simulink model "mavsim"  (R2025b)
settings: Solver=ode45  StartTime=0.0  StopTime=80  RelTol=1e-3
undefined symbols (not defined in the file): animation_block, autopilot_block, forces_block, P, wind_block
settings Model: Creator=parakh  LastModifiedBy=parakh

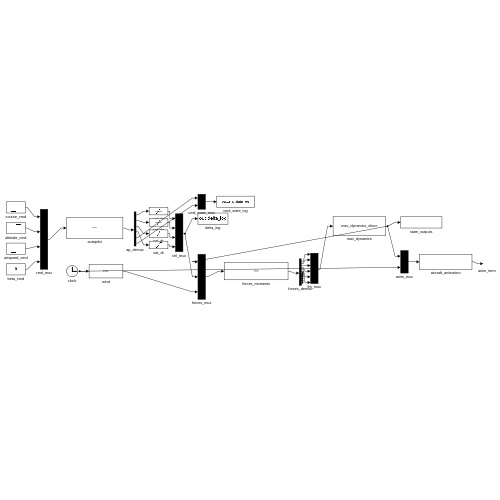
[thumbnail: Simulink's stored preview of the top-level diagram]
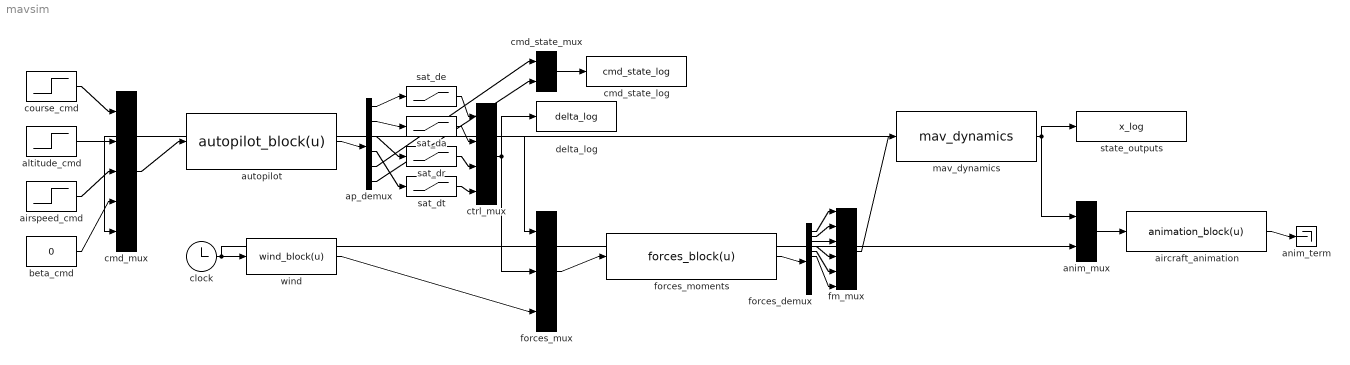
== system mavsim ==
  aircraft_animation : MATLABFcn  MATLABFcn=animation_block(u)  OutputDimensions=1
  airspeed_cmd : Step  Time=45  Before=25  After=27  SampleTime=0
  altitude_cmd : Step  Time=25  Before=100  After=110  SampleTime=0
  anim_mux : Mux  Inputs=2
  anim_term : Terminator
  ap_demux : Demux  Outputs=6
  autopilot : MATLABFcn  MATLABFcn=autopilot_block(u)  OutputDimensions=6
  beta_cmd : Constant  Value=0
  clock : Clock
  cmd_mux : Mux  Inputs=5
  cmd_state_log : ToWorkspace  VariableName=cmd_state_log  SampleTime=-1
  cmd_state_mux : Mux  Inputs=2
  course_cmd : Step  Time=10  After=15*pi/180  SampleTime=0
  ctrl_mux : Mux
  delta_log : ToWorkspace  VariableName=delta_log  SampleTime=-1
  fm_mux : Mux  Inputs=6
  forces_demux : Demux  Outputs=12
  forces_moments : MATLABFcn  MATLABFcn=forces_block(u)  OutputDimensions=12
  forces_mux : Mux  Inputs=3
  mav_dynamics : M-S-Function  FunctionName=mav_dynamics  Parameters=P
  sat_da : Saturate  UpperLimit=P.delta_a_max  LowerLimit=-P.delta_a_max
  sat_de : Saturate  UpperLimit=P.delta_e_max  LowerLimit=-P.delta_e_max
  sat_dr : Saturate  UpperLimit=P.delta_r_max  LowerLimit=-P.delta_r_max
  sat_dt : Saturate  UpperLimit=P.delta_t_max  LowerLimit=P.delta_t_min
  state_outputs : ToWorkspace  VariableName=x_log  SampleTime=-1
  wind : MATLABFcn  MATLABFcn=wind_block(u)  OutputDimensions=6
  wires:
  course_cmd/1 -> cmd_mux/1
  altitude_cmd/1 -> cmd_mux/2
  airspeed_cmd/1 -> cmd_mux/3
  beta_cmd/1 -> cmd_mux/4
  cmd_mux/1 -> autopilot/1
  autopilot/1 -> ap_demux/1
  ap_demux/1 -> sat_de/1
  ap_demux/2 -> sat_da/1
  ap_demux/3 -> sat_dr/1
  ap_demux/4 -> sat_dt/1
  sat_de/1 -> ctrl_mux/1
  sat_da/1 -> ctrl_mux/2
  sat_dr/1 -> ctrl_mux/3
  sat_dt/1 -> ctrl_mux/4
  ctrl_mux/1 -> delta_log/1, forces_mux/2
  ap_demux/5 -> cmd_state_mux/1
  ap_demux/6 -> cmd_state_mux/2
  cmd_state_mux/1 -> cmd_state_log/1
  clock/1 -> wind/1, anim_mux/2
  mav_dynamics/1 -> forces_mux/1, state_outputs/1, anim_mux/1, cmd_mux/5
  wind/1 -> forces_mux/3
  forces_mux/1 -> forces_moments/1
  forces_moments/1 -> forces_demux/1
  forces_demux/1 -> fm_mux/1
  forces_demux/2 -> fm_mux/2
  forces_demux/3 -> fm_mux/3
  forces_demux/4 -> fm_mux/4
  forces_demux/5 -> fm_mux/5
  forces_demux/6 -> fm_mux/6
  fm_mux/1 -> mav_dynamics/1
  anim_mux/1 -> aircraft_animation/1
  aircraft_animation/1 -> anim_term/1
